simulink model "MATE_PMSMDynamicSwitches"  (R2024b)
settings: Solver=FixedStepDiscrete  StartTime=0.0  StopTime=0.6  RelTol=1e-3  AbsTol=1e-3
PreLoadFcn:
  | % Control parameters
  | Ts = 2e-6;   % Fundamental sample time
  | fsw = 2e3;   % Switching frequency (Hz)
  | fc = fsw*10; % Control loop frequency (Hz)
  | Tsc = 1/fc;  % Control loop sample time
  | 
  | % PMSM parameters
  | PM = 0.03; % Permanent magnet flux linkage
  | Ld = 2e-4;  % d-axis inductance
  | Lq = 2e-4;  % q-axis inductance
  | L0 = 2e-4;  % 0-axis inductance
  | Rs = 0.013; % Stator resistance
  | N = 6; % Number of pole pairs
  | J = 0.2; % Moment of inertia
  | 
  | % Operating and derived limits
  | Imax = 100;  % Max stator current (peak value)
  | Tmax = 1.5*N*PM*Imax; % Max lectromagnetic torque
  | fnom = 100;  % Nominal frequency (Hz)
  | rpm_nom = 60*fnom/N;      % Nominal rotor speed (rpm)
  | omegam_nom = 2*pi*fnom/N; % Nominal mechanical rotor speed
  | Pmax = omegam_nom*Tmax;     % Maximum power
  | 
  | Gs = 4.4526;
  | s = 2.8994;
  | h = 2e-6;
InitFcn:
  | % Control parameters
  | Ts = 2e-6;   % Fundamental sample time
  | fsw = 2e3;   % Switching frequency (Hz)
  | fc = fsw*10; % Control loop frequency (Hz)
  | Tsc = 1/fc;  % Control loop sample time
  | 
  | % PMSM parameters
  | PM = 0.03; % Permanent magnet flux linkage
  | Ld = 2e-4;  % d-axis inductance
  | Lq = 2e-4;  % q-axis inductance
  | L0 = 2e-4;  % 0-axis inductance
  | Rs = 0.013; % Stator resistance
  | N = 6; % Number of pole pairs
  | J = 0.2; % Moment of inertia
  | 
  | % Operating and derived limits
  | Imax = 100;  % Max stator current (peak value)
  | Tmax = 1.5*N*PM*Imax; % Max lectromagnetic torque
  | fnom = 100;  % Nominal frequency (Hz)
  | rpm_nom = 60*fnom/N;      % Nominal rotor speed (rpm)
  | omegam_nom = 2*pi*fnom/N; % Nominal mechanical rotor speed
  | Pmax = omegam_nom*Tmax;     % Maximum power
  | 
  | Gs = 4.4526;
  | s = 2.8994;
  | h = 2e-6;
libraries: nesl_utility x7, fl_lib x6, simetranss x3, ee_lib x3, batteryecm_lib x1, eePmsmFieldOrientedControl x1
Description:
  | Three-Phase PMSM Drive
settings Model: DataTypeOverride=Off  Creator=Kyle Diller
settings SolverCC: AutoScaleAbsTol=off  MaxConsecutiveMinStep=2  ZeroCrossAlgorithm=Adaptive  AlgebraicLoopSolver=TrustRegion  MaxZcPerStep=1
settings DataIOCC: LimitDataPoints=on  MaxDataPoints=690000  SaveFormat=Array  ReturnWorkspaceOutputs=off  SignalLoggingName=logsout_ee_pmsm_drive
settings OptimizationCC: BlockReduction=off  ConditionallyExecuteInputs=off  DefaultParameterBehavior=Inlined  InheritOutputTypeSmallerThanSingle=on  ReuseModelBlockBuffer=off  LifeSpan=inf
settings DebuggingCC: AlgebraicLoopMsg=error  MaxConsecutiveZCsMsg=none  IgnoredZcDiagnostic=none  SingleTaskRateTransMsg=error  UnconnectedInputMsg=warning  UnconnectedOutputMsg=warning  UnconnectedLineMsg=warning  AllowSymbolicDim=off  PregeneratedLibrarySubsystemCodeDiagnostic=none  SFUnexpectedBacktrackingDiag=warning  SFNoUnconditionalDefaultTransitionDiag=warning  SFExecutionAtInitializationDiag=none  ArithmeticOperatorsInVariantConditions=warning
settings HardwareCC: ProdBitPerPointer=32  ProdBitPerSizeT=32  ProdBitPerPtrDiffT=32  ProdLargestAtomicFloat=None  ProdIntDivRoundTo=Undefined  ProdEndianess=Unspecified  ProdWordSize=32  ProdHWDeviceType=ASIC/FPGA->ASIC/FPGA  TargetBitPerPointer=64  TargetBitPerSizeT=64  TargetBitPerPtrDiffT=64  TargetLongLongMode=on  TargetIntDivRoundTo=Zero  TargetEndianess=LittleEndian  TargetWordSize=64  TargetHWDeviceType=Custom Processor->MATLAB Host Computer  ProdEqTarget=off
settings ModelReferenceCC: EnableRefExpFcnMdlSchedulingChecks=on  PropagateSignalLabelsOutOfModel=off
settings SFSimCC: SimUseLocalCustomCode=off
settings RTWCC: RTWUseLocalCustomCode=off  GPUComputeCapability=3.5  DLArmComputeVersion=19.05
settings CodeAppCC: StateflowObjectComments=on
settings GRTTargetCC: TargetLangStandard=C89/C90 (ANSI)
settings ConfigComp: CovMetricSettings=dw  CovSaveCumulativeToWorkspaceVar=on  CovSaveSingleToWorkspaceVar=on  CovExternalEMLEnable=off  CovSFcnEnable=off
settings SimscapeCC: SimscapeLogType=all  SimscapeLogSimulationStatistics=on  SimscapeLogName=simlog_ee_pmsm_drive  SimscapeLogDataHistory=690000

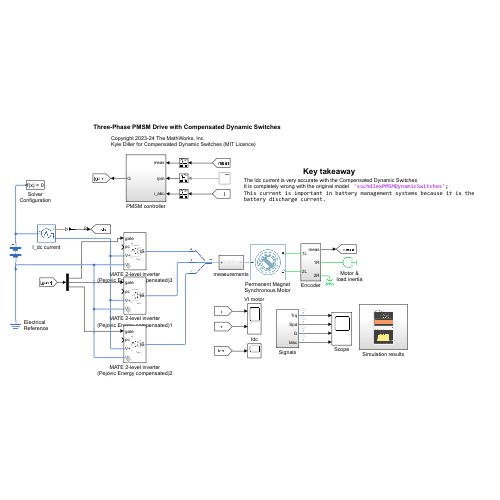
[thumbnail: Simulink's stored preview of the top-level diagram]
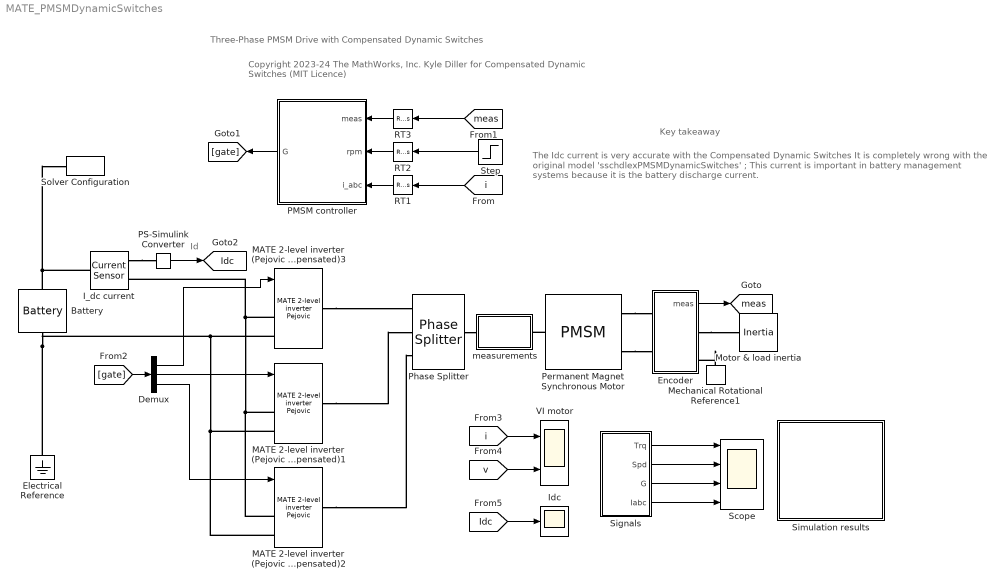
== system MATE_PMSMDynamicSwitches ==
  note: Key takeaway
  note: The Idc current is very accurate with the Compensated Dynamic Switches
      | It is completely wrong with the original model 'sschdlexPMSMDynamicSwitches' ;
      | This current is important in battery management systems because it is the battery discharge current.
  note: Id
  note: Three-Phase PMSM Drive with Compensated Dynamic Switches
  note: Copyright 2023-24 The MathWorks, Inc.
      | Kyle Diller for Compensated Dynamic Switches (MIT Licence)
  Battery : batteryecm_lib/Battery  Vnom=48 V  prm_dir=1  R1_dis=2 Ohm  R1_ch=2 Ohm  R1=0.001 Ohm  prm_AH=1  AH=14000 hr*A  V1=470 V  AH1=5000 hr*A  prm_R2=1  R2=inf Ohm  Tmeas=298.15 K  charge_measurement_port=simscape.enum.battery.enable.no  prm_dyn=1  Rp1=0.005 Ohm  tau1=30 s  Rp2=0.005 Ohm  tau2=30 s  Rp3=0.005 Ohm  tau3=30 s  Rp4=0.005 Ohm  tau4=30 s  Rp5=0.005 Ohm  tau5=30 s  prm_fade=1  N_fade=100  AH_fade=45 hr*A  R1_fade=2.02 Ohm  R1_ch_fade=2.02 Ohm  V1_fade=10.35 V  prm_age=1  prm_age_OCV=1  OCV_age=0.9  SOC_age=60  Tmeas_age=298.15 K  delta_time_age_vec=[0] d  temperature_age_vec=[273] K  OCV_scaling_age=2.2134e6  OCV_offset_age=1.632e6  temp_exp_age=0.515833569 V  t_exp_age=0.75  Vnom_T2=12 V  R1_T2=2.2 Ohm  R1_T2_dis=2.2 Ohm  R1_T2_ch=2.2 Ohm  V1_T2=11.4 V  R2_T2=2200 Ohm  Rp1_T2=0.005 Ohm  tau1_T2=30 s  Rp2_T2=0.005 Ohm  tau2_T2=30 s  Rp3_T2=0.005 Ohm  tau3_T2=30 s  Rp4_T2=0.005 Ohm  tau4_T2=30 s  Rp5_T2=0.005 Ohm  tau5_T2=30 s  Tmeas2=273.15 K  thermal_port=simscape.enum.thermaleffects.omit  thermal_mass=30000 J/K  i_specify=off  i_priority=None  i=0 A  i_nominal_specify=off  i_nominal_value=1  i_nominal_unit=A  v_specify=off  v_priority=None  v=0 V  v_nominal_specify=off  v_nominal_value=1  v_nominal_unit=V  charge_specify=on  charge_priority=High  charge=7000 hr*A  charge_nominal_specify=off  charge_nominal_value=1  charge_nominal_unit=A*hr  num_cycles_specify=off  num_cycles_priority=High  num_cycles=0  num_cycles_nominal_specify=off  num_cycles_nominal_value=1  num_cycles_nominal_unit=1  temperature_specify=off  temperature_priority=High  temperature=298.15 K  temperature_nominal_specify=off  temperature_nominal_value=1  temperature_nominal_unit=K
  Demux : Demux  Outputs=[2 2 2]
  Electrical Reference : fl_lib/Electrical/Electrical Elements/Electrical Reference
  Encoder : Subsystem
  I_dc current : fl_lib/Electrical/Electrical Sensors/Current Sensor
  Idc : Scope
  MATE 2-level inverter (Pejovic Energy compensated)1 : simetranss/FPGA/MATE 2-level inverter Pejovic  Lon=1e-6  Ts=Ts
  MATE 2-level inverter (Pejovic Energy compensated)2 : simetranss/FPGA/MATE 2-level inverter Pejovic  Lon=1e-6  Ts=Ts
  MATE 2-level inverter (Pejovic Energy compensated)3 : simetranss/FPGA/MATE 2-level inverter Pejovic  Lon=1e-6  Ts=Ts
  Mechanical Rotational Reference1 : fl_lib/Mechanical/Rotational Elements/Mechanical Rotational Reference
  Motor & load inertia : fl_lib/Mechanical/Rotational Elements/Inertia  inertia=J kg*m^2  num_ports=foundation.enum.numPorts2.one  w_specify=on  w_priority=High  w=0 rpm  w_nominal_specify=off  w_nominal_value=1  w_nominal_unit=rad/s  t_specify=off  t_priority=High  t=0 N*m  t_nominal_specify=off  t_nominal_value=1  t_nominal_unit=N*m
  PMSM controller : Subsystem
  PS-Simulink Converter : nesl_utility/PS-Simulink Converter  PhysicalDomain=network_engine_domain  SubClassName=ps_output  LeftPortType=input  RightPortType=output  PseudoPeriodic=off  Frequencies=[]  VectorFormat=inherit  Unit=inherit  AffineConversion=off
  Permanent Magnet Synchronous Motor : ee_lib/Electromechanical/Permanent Magnet/PMSM  port_option=ee.enum.threePhasePort.composite  winding_type=ee.enum.statorconnection.wye  machine_param=ee.enum.pmsm.parameterization.constant  nPolePairs=N  pmflux_param=ee.enum.pmflux.fluxlinkage  pm_flux_linkage=PM Wb  torque_constant=0.18 N*m/A  back_emf_constant=0.18 V/(rad/s)  stator_param=ee.enum.statorparam.LdLqL0  Ld=Ld H  Lq=Lq H  idVec=[-200, 0, 200] A  iqVec=[-200, 0, 200] A  LdMatrix=0.0002 * ones(3, 3) H  LqMatrix=0.0002 * ones(3, 3) H  PmMatrix=0.1 * ones(3, 3) Wb  ktMatrix=0.18 * ones(3, 3) N*m/A  keMatrix=0.18 * ones(3, 3) V/(rad/s)  L0=L0 H  Ls=0.0002 H  Lm=0.00002 H  Ms=0.00002 H  Rs=Rs Ohm  zero_sequence=ee.enum.park.zerosequence.exclude  axes_param=ee.enum.rotorangle.qaxis  loss_param=ee.enum.ironloss.none  losses_oc=[0, 0, 0] W  losses_sc=[0, 0, 0] W  f_losses=60 Hz  Isc_losses=95 A  J=0 kg*m^2  lam=0 N*m/(rad/s)  i_d_specify=off  i_d_priority=None  i_d=0 A  i_d_nominal_specify=off  i_d_nominal_value=1  i_d_nominal_unit=A  i_q_specify=off  i_q_priority=None  i_q=0 A  i_q_nominal_specify=off  i_q_nominal_value=1  i_q_nominal_unit=A  torque_specify=off  torque_priority=None  torque=0 N*m  torque_nominal_specify=off  torque_nominal_value=1  torque_nominal_unit=N*m  angular_velocity_specify=on  angular_velocity_priority=None  angular_velocity=0 rpm  angular_velocity_nominal_specify=off  angular_velocity_nominal_value=1  angular_velocity_nominal_unit=rpm  angular_position_specify=on  angular_position_priority=High  angular_position=0 rad  angular_position_nominal_specify=off  angular_position_nominal_value=1  angular_position_nominal_unit=deg  alpha=3.93e-3 1/K  alpha_flux=-0.001 1/K  Tmeas=298.15 K  stator_thermal_mass=100 J/K  rotor_thermal_mass=200 J/K  Rm_percent_rotor=90  Rd_percent_rotor=30  temperatureA_specify=off  temperatureA_priority=High  temperatureA=25 degC  temperatureA_nominal_specify=off  temperatureA_nominal_value=1  temperatureA_nominal_unit=degC  temperatureB_specify=off  temperatureB_priority=High  temperatureB=25 degC  temperatureB_nominal_specify=off  temperatureB_nominal_value=1  temperatureB_nominal_unit=degC  temperatureC_specify=off  temperatureC_priority=High  temperatureC=25 degC  temperatureC_nominal_specify=off  temperatureC_nominal_value=1  temperatureC_nominal_unit=degC  temperatureR_specify=off  temperatureR_priority=High  temperatureR=25 degC  temperatureR_nominal_specify=off  temperatureR_nominal_value=1  temperatureR_nominal_unit=degC
      settings: InternalSimscapePortConfiguration="{\"Bottom\":[],\"Left\":[{\"id\":\"N\",\"label\":\"~\",\"type\":\"foundation.electrical.three_phase\"}],\"Right\":[{\"id\":\"R\",\"label\":\"R\",\"type\":\"foundation.mechanical.rotational.rotational\"},{\"id\":\"C\",\"label\":\"C\",\"type\":\"foundation.mechanical.rotational.rotational\"}],\"Top\":[]}"
  Phase Splitter : ee_lib/Connectors & References/Phase Splitter
  RT1 : RateTransition  OutPortSampleTime=Tsc
  RT2 : RateTransition  OutPortSampleTime=Tsc
  RT3 : RateTransition  OutPortSampleTime=Tsc
  Scope : Scope  NumInputPorts=4
  "Signals " : Subsystem
  Simulation results : Subsystem
  Solver Configuration : nesl_utility/Solver Configuration  PhysicalDomain=network_engine_domain  SubClassName=solver  LeftPortType=input  RightPortType=generic  Tones=[]  Harmonics=[]  SimulateNoise=off  Profile=off  UseLocalSampling=off  EnableSwitchedLinearOptims=on  FrequencyDomain=off  UseCCode=off  RelTol=0.001  AbsTol=1e-06  MinStep=1e-09  ToWorkspace=off  RevertToSquareIcSolve=off  NumHomotopyIterations=100  PhasorMode=off  PhasorModeNumHarmonics=1  ConsistencySolver=NEWTON_FTOL  IndexReductionMethod=DerivativeReplacement  DoDC=off  ResidualTolerance=1e-9  ConsistencyTolSource=GLOBAL  ConsistencyAbsTol=0.001  ConsistencyRelTol=0.001  ConsistencyTolFactor=0.001  UseLocalSolver=on  LocalSolverChoice=NE_PARTITIONING_ADVANCER  ResolveIndetEquations=on  FunctionEvalNumThread=1  LocalSolverSampleTime=Ts  DoFixedCost=on  MaxNonlinIter=4  MaxModeIter=2  ComputeImpulses=off  ImpulseIterations=2  LinearAlgebra=auto  LinearAlgebraNumThread=0  EquationFormulation=NE_TIME_EF  DelaysMemoryBudget=1024  AutomaticFiltering=on  FilteringTimeConstant=0.001  PartitionStorageMethod=AS_NEEDED  PartitionMemoryBudget=1024  PartitionMethod=FAST  MultibodyUseLocalSolver=off  MultibodyLocalSolverChoice=ODE1  MultibodyLocalSolverSampleTime=0.001
  Step : Step  Time=0.1  After=500  SampleTime=0
  VI motor : Scope  NumInputPorts=2
  measurements : Subsystem
  tag scope: Idc=global, meas=global
  wires:
  Step/1 -> RT2/1
  RT3/1 -> PMSM controller/1(meas)
  RT2/1 -> PMSM controller/2(rpm)
  RT1/1 -> PMSM controller/3(i_abc)
  "Signals "/2(Spd) -> Scope/2
  "Signals "/4(Iabc) -> Scope/4
  "Signals "/3(G) -> Scope/3
  "Signals "/1(Trq) -> Scope/1
  [i] -> RT1/1
  Encoder/1(meas) -> [meas]
  [meas] -> RT3/1
  PMSM controller/1(G) -> [gate]
  Demux/2 -> MATE 2-level inverter (Pejovic Energy compensated)1/1
  Demux/1 -> MATE 2-level inverter (Pejovic Energy compensated)3/1
  Demux/3 -> MATE 2-level inverter (Pejovic Energy compensated)2/1
  [gate] -> Demux/1
  [i] -> VI motor/1
  [v] -> VI motor/2
  PS-Simulink Converter/1 -> [Idc]
  [Idc] -> Idc/1
  connections:
  Battery/LConn1 -- I_dc current/LConn1 -- Solver Configuration/RConn1
  Permanent Magnet Synchronous Motor/RConn1 -- Encoder/LConn1
  Permanent Magnet Synchronous Motor/RConn2 -- Encoder/LConn2
  Encoder/RConn1 -- Motor & load inertia/LConn1
  Mechanical Rotational Reference1/LConn1 -- Encoder/RConn2
  Electrical Reference/LConn1 -- MATE 2-level inverter (Pejovic Energy compensated)3/LConn2 -- MATE 2-level inverter (Pejovic Energy compensated)2/LConn2 -- MATE 2-level inverter (Pejovic Energy compensated)1/LConn2 -- Battery/RConn1
  I_dc current/RConn1 -- PS-Simulink Converter/LConn1
  I_dc current/RConn2 -- MATE 2-level inverter (Pejovic Energy compensated)3/LConn1 -- MATE 2-level inverter (Pejovic Energy compensated)2/LConn1 -- MATE 2-level inverter (Pejovic Energy compensated)1/LConn1
  MATE 2-level inverter (Pejovic Energy compensated)3/RConn1 -- Phase Splitter/RConn1
  MATE 2-level inverter (Pejovic Energy compensated)1/RConn1 -- Phase Splitter/RConn2
  MATE 2-level inverter (Pejovic Energy compensated)2/RConn1 -- Phase Splitter/RConn3
  Phase Splitter/LConn1 -- measurements/LConn1
  Permanent Magnet Synchronous Motor/LConn1 -- measurements/RConn1

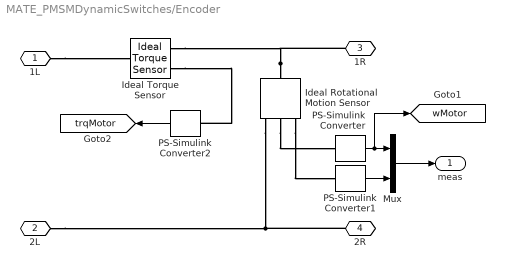
== system MATE_PMSMDynamicSwitches/Encoder ==
  Ideal Rotational Motion Sensor : fl_lib/Mechanical/Mechanical Sensors/Ideal Rotational Motion Sensor  reference=foundation.enum.MeasurementReference.difference  acceleration_port=false  velocity_port=true  position_port=true  wrap_angle=simscape.enum.onoff.off  offset=0 deg
  Ideal Torque Sensor : fl_lib/Mechanical/Mechanical Sensors/Ideal Torque Sensor
  Mux : Mux  Inputs=2
  PS-Simulink Converter : nesl_utility/PS-Simulink Converter  PhysicalDomain=network_engine_domain  SubClassName=ps_output  LeftPortType=input  RightPortType=output  PseudoPeriodic=off  Frequencies=[]  VectorFormat=1-D array  Unit=rad/s  AffineConversion=off
  PS-Simulink Converter1 : nesl_utility/PS-Simulink Converter  PhysicalDomain=network_engine_domain  SubClassName=ps_output  LeftPortType=input  RightPortType=output  PseudoPeriodic=off  Frequencies=[]  VectorFormat=1-D array  Unit=rad  AffineConversion=off
  PS-Simulink Converter2 : nesl_utility/PS-Simulink Converter  PhysicalDomain=network_engine_domain  SubClassName=ps_output  LeftPortType=input  RightPortType=output  PseudoPeriodic=off  Frequencies=[]  VectorFormat=1-D array  Unit=N*m  AffineConversion=off
  1L : PMIOPort  Side=Left
  2L : PMIOPort  Port=2  Side=Left
  1R : PMIOPort  Port=3  Side=Right
  2R : PMIOPort  Port=4  Side=Right
  meas : Outport  VectorParamsAs1DForOutWhenUnconnected=off
  tag scope: trqMotor=global, wMotor=global
  wires:
  PS-Simulink Converter2/1 -> [trqMotor]
  Mux/1 -> meas/1
  PS-Simulink Converter1/1 -> Mux/2
  PS-Simulink Converter/1 -> [wMotor], Mux/1
  connections:
  Ideal Torque Sensor/RConn2 -- PS-Simulink Converter2/LConn1
  1L/RConn1 -- Ideal Torque Sensor/LConn1
  2R/RConn1 -- 2L/RConn1 -- Ideal Rotational Motion Sensor/RConn1
  Ideal Rotational Motion Sensor/LConn1 -- 1R/RConn1 -- Ideal Torque Sensor/RConn1
  Ideal Rotational Motion Sensor/RConn2 -- PS-Simulink Converter/LConn1
  Ideal Rotational Motion Sensor/RConn3 -- PS-Simulink Converter1/LConn1

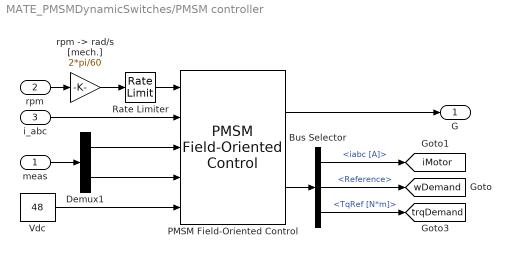
== system MATE_PMSMDynamicSwitches/PMSM controller ==
  meas : Inport
  rpm : Inport  Port=2
  i_abc : Inport  Port=3
  Bus Selector : BusSelector  OutputSignals=iabc [A],Reference,TqRef [N*m]
  Demux1 : Demux  Outputs=2
  PMSM Field-Oriented Control : eePmsmFieldOrientedControl/PMSM Field-Oriented Control  winding_type=Wye-wound  CtrlMode=Velocity control  Vnom=48  Pmax=Pmax  Tmax=Tmax*1.5  p=N  Vdc_on=10  Ts=Ts  Tsc=Tsc  CtrlType=PI control  Kp_w=60  Ki_w=300*2  Kv_w=1  Kaw_w=1000  RefType=Zero d-axis control  rpmVec=[0, 3000]  TqVec=[-100, 0, 100]  VdcVec=[300, 350]  PWMMode=SPWM: sinusoidal PWM  ModFactor=1  idMatrix=zeros(2,3,2)  iqMatrix=zeros(2,3,2)  psim=PM  Ld=0.00024  Lq=0.00029  Rs=0.01  AxisAlignment=Q-axis  Kp_id=0.1  Ki_id=10  Kaw_id=1000  Kp_iq=0.1  Ki_iq=10  Kaw_iq=1000  AxisPrio=Q-axis  ActZC=off  ActFF=on  ParamTypeFF=Constant parameters  LdFF=Ld  LqFF=Lq  psimFF=PM  idVect=[-200, 0, 200]  iqVect=[-200, 0, 200]  LdMatrix=0.0002 * ones(3, 3)  LqMatrix=0.0002 * ones(3, 3)  psimMatrix=0.04 * ones(3, 3)  CPWMMode=SPWM: sinusoidal PWM  fsw=fsw
  Rate Limiter : RateLimiter  RisingSlewLimit=Tmax/J  FallingSlewLimit=-Tmax/J  SampleTimeMode=inherited
  Vdc : Constant  Value=48  SampleTime=Tsc
  "rpm -> rad/s [mech.]" : Gain  Gain=2*pi/60
  G : Outport  VectorParamsAs1DForOutWhenUnconnected=off
  tag scope: iMotor=global, trqDemand=global, wDemand=global
  wires:
  PMSM Field-Oriented Control/1 -> G/1
  Vdc/1 -> PMSM Field-Oriented Control/5
  PMSM Field-Oriented Control/2 -> Bus Selector/1
  i_abc/1 -> PMSM Field-Oriented Control/2
  meas/1 -> Demux1/1
  Demux1/1 -> PMSM Field-Oriented Control/3
  Demux1/2 -> PMSM Field-Oriented Control/4
  Bus Selector/1 -> [iMotor]  "<iabc [A]>"
  Bus Selector/2 -> [wDemand]  "<Reference>"
  Bus Selector/3 -> [trqDemand]  "<TqRef [N*m]>"
  rpm/1 -> "rpm -> rad/s [mech.]"/1
  Rate Limiter/1 -> PMSM Field-Oriented Control/1
  "rpm -> rad/s [mech.]"/1 -> Rate Limiter/1

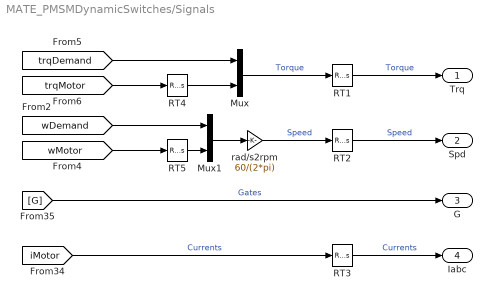
== system MATE_PMSMDynamicSwitches/Signals  ==
  Mux : Mux  Inputs=2
  Mux1 : Mux  Inputs=2
  RT1 : RateTransition  OutPortSampleTime=Ts
  RT2 : RateTransition  OutPortSampleTime=Ts
  RT3 : RateTransition  OutPortSampleTime=Ts
  RT4 : RateTransition  OutPortSampleTime=Tsc
  RT5 : RateTransition  OutPortSampleTime=Tsc
  rad/s2rpm : Gain  Gain=60/(2*pi)
  Trq : Outport  VectorParamsAs1DForOutWhenUnconnected=off
  Spd : Outport  Port=2  VectorParamsAs1DForOutWhenUnconnected=off
  G : Outport  Port=3  VectorParamsAs1DForOutWhenUnconnected=off
  Iabc : Outport  Port=4  VectorParamsAs1DForOutWhenUnconnected=off
  wires:
  [trqDemand] -> Mux/1
  [G] -> G/1  "Gates"
  Mux1/1 -> rad/s2rpm/1
  Mux/1 -> RT1/1  "Torque"
  [iMotor] -> RT3/1  "Currents"
  [wDemand] -> Mux1/1
  rad/s2rpm/1 -> RT2/1  "Speed"
  [trqMotor] -> RT4/1
  [wMotor] -> RT5/1
  RT1/1 -> Trq/1  "Torque"
  RT2/1 -> Spd/1  "Speed"
  RT3/1 -> Iabc/1  "Currents"
  RT4/1 -> Mux/2
  RT5/1 -> Mux1/2

== system MATE_PMSMDynamicSwitches/Simulation results ==
  note: df
  note: f g

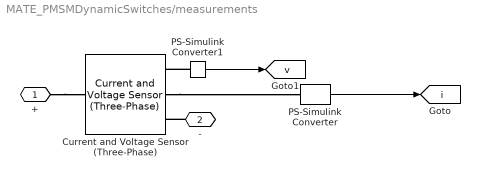
== system MATE_PMSMDynamicSwitches/measurements ==
  Current and Voltage Sensor (Three-Phase) : ee_lib/Sensors & Transducers/Current and Voltage Sensor (Three-Phase)  vMeasurementType=ee.enum.vmeasurement.lg  outputUnit=ee.enum.unit.si  SRated=100e6 A*V  VRated=24e3 V  I_specify=off  I_priority=None  I=[0, 0, 0] A  I_nominal_specify=off  I_nominal_value=1  I_nominal_unit=A  V_specify=off  V_priority=None  V=[0, 0, 0] V  V_nominal_specify=off  V_nominal_value=1  V_nominal_unit=V
      settings: InternalSimscapePortConfiguration="{\"Bottom\":[],\"Left\":[{\"id\":\"N1\",\"label\":\"~1\",\"type\":\"foundation.electrical.three_phase\"}],\"Right\":[{\"id\":\"V_output\",\"label\":\"V\",\"type\":\"output\"},{\"id\":\"I_output\",\"label\":\"I\",\"type\":\"output\"},{\"id\":\"N2\",\"label\":\"~2\",\"type\":\"foundation.electrical.three_phase\"}],\"Top\":[]}"
  PS-Simulink Converter : nesl_utility/PS-Simulink Converter  PhysicalDomain=network_engine_domain  SubClassName=ps_output  LeftPortType=input  RightPortType=output  PseudoPeriodic=off  Frequencies=[]  VectorFormat=1-D array  Unit=A  AffineConversion=off
  PS-Simulink Converter1 : nesl_utility/PS-Simulink Converter  PhysicalDomain=network_engine_domain  SubClassName=ps_output  LeftPortType=input  RightPortType=output  PseudoPeriodic=off  Frequencies=[]  VectorFormat=inherit  Unit=inherit  AffineConversion=off
  + : PMIOPort  Side=Left
  - : PMIOPort  Port=2  Side=Right
  tag scope: i=global, v=global
  wires:
  PS-Simulink Converter1/1 -> [v]
  PS-Simulink Converter/1 -> [i]
  connections:
  PS-Simulink Converter1/LConn1 -- Current and Voltage Sensor (Three-Phase)/RConn1
  +/RConn1 -- Current and Voltage Sensor (Three-Phase)/LConn1
  -/RConn1 -- Current and Voltage Sensor (Three-Phase)/RConn3
  Current and Voltage Sensor (Three-Phase)/RConn2 -- PS-Simulink Converter/LConn1
